simulink model "tcp_gantry_logic"  (R2025b)
settings: Solver=FixedStepAuto  StartTime=0.0  StopTime=inf  RelTol=1e-3  EnableMultiTasking=on
libraries: simulink x4, raspberrypiNetworklib x1
settings Model: ExtModeTrigDuration=2  Creator=rico_jitin  LastModifiedBy=rico_jitin
settings SolverCC: PositivePriorityOrder=on
settings OptimizationCC: EnhancedBackFolding=on  PassReuseOutputArgsAs=Individual arguments  ZeroExternalMemoryAtStartup=off  ZeroInternalMemoryAtStartup=off  MaxStackSize=200000  OptimizeBlockOrder=speed  DifferentSizesBufferReuse=on  OptimizationCustomize=off  EfficientTunableParamExpr=on
settings DebuggingCC: ParameterTunabilityLossMsg=error
settings HardwareCC: ProdBitPerPointer=32.0  ProdBitPerSizeT=32.0  ProdBitPerPtrDiffT=32.0  ProdLargestAtomicInteger=Long  ProdLargestAtomicFloat=Double  ProdWordSize=32.0  ProdLongLongMode=on  ProdHWDeviceType=ARM Compatible->ARM Cortex-A (32-bit)
settings RTWCC: SystemTargetFile=ert.tlc  HardwareBoard=Raspberry Pi  TLCOptions="-aInlineSetEventsForThisBaseRateFcn=TLC_FALSE -aSuppressMultiTaskScheduler=TLC_FALSE  -aRateBasedStepFcn=0"  TemplateMakefile=ert_default_tmf  Toolchain=GNU GCC Embedded Linux  BuildConfiguration=Faster Runs  Description=Embedded Coder
settings CodeAppCC: ForceParamTrailComments=on  IgnoreCustomStorageClasses=off  OperatorAnnotations=on  SimulinkDataObjDesc=on  SFDataObjDesc=on  InsertBlockDesc=on
settings ERTTargetCC: ExtModeTransport=2.0  ExtModeStaticAlloc=on  ExtModeMexFile=ext_xcp  ExtModeIntrfLevel=Level2 - Open  InlinedParameterPlacement=Hierarchical  CodeReplacementLibrary=ARM Cortex-A CMSIS  SupportVariableSizeSignals=on

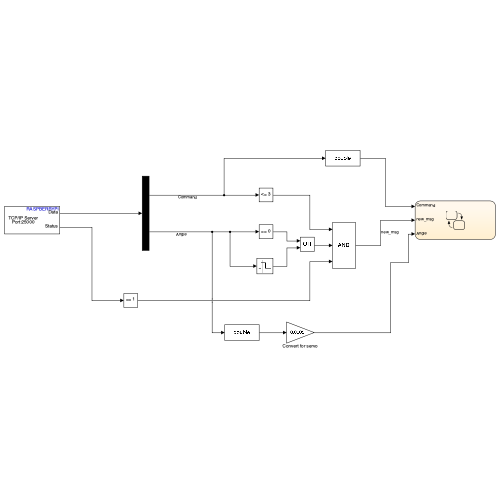
[thumbnail: Simulink's stored preview of the top-level diagram]
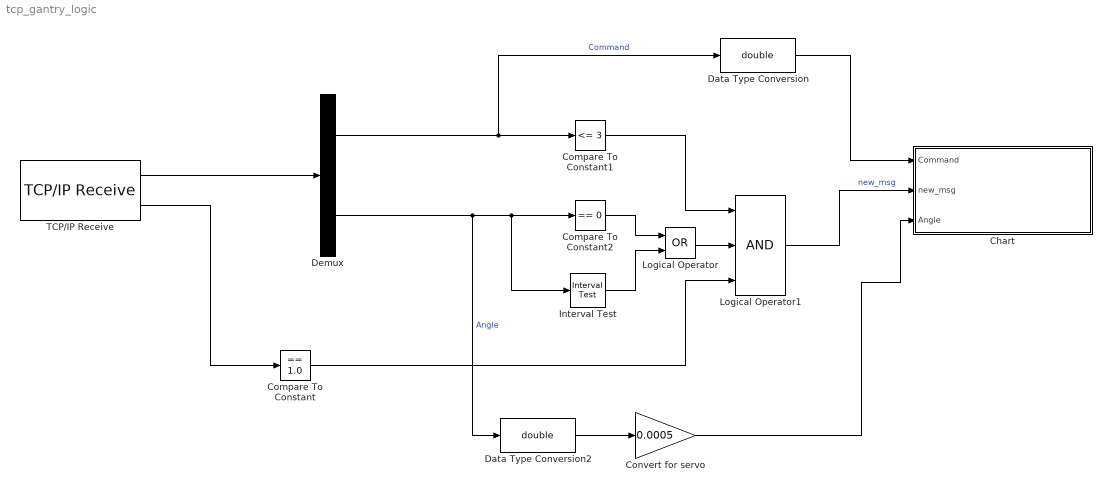
== system tcp_gantry_logic ==
  Chart : Stateflow chart  TreatAsAtomicUnit=on
  Compare To Constant : simulink/Logic and Bit Operations/Compare To Constant  relop===  const=1.0  OutDataTypeStr=boolean
  Compare To Constant1 : simulink/Logic and Bit Operations/Compare To Constant  relop=<=  const=3  OutDataTypeStr=boolean
  Compare To Constant2 : simulink/Logic and Bit Operations/Compare To Constant  relop===  const=0  OutDataTypeStr=boolean
  Convert for servo : Gain  Gain=0.0005
  Data Type Conversion : DataTypeConversion  OutDataTypeStr=double  SaturateOnIntegerOverflow=off  RndMeth=Floor
  Data Type Conversion2 : DataTypeConversion  OutDataTypeStr=double  SaturateOnIntegerOverflow=off  RndMeth=Floor
  Demux : Demux  Outputs=2
  Interval Test : simulink/Logic and Bit Operations/Interval Test  IntervalClosedRight=on  uplimit=200  IntervalClosedLeft=on  lowlimit=100  OutDataTypeStr=boolean
  Logical Operator : Logic  Operator=OR  AllPortsSameDT=off  OutDataTypeStr=boolean
  Logical Operator1 : Logic  Inputs=3  AllPortsSameDT=off  OutDataTypeStr=boolean
  TCP/IP Receive : raspberrypiNetworklib/TCP//IP Receive  Mode_=Server  LocalServerPort_=25000  RemoteAddr_=127.0.0.1  RemoteServerPort_=25000  DataType_=uint8  DataSize_=2  SampleTime_=0.002  SimulateUsing=Code generation  ClientPortBindingSelection_=off  ClientPortToBind_=35000  BlockingMode_=off  BlockTimeout_=0.1  BlockPlatform=RASPBERRYPI
  wires:
  TCP/IP Receive/1 -> Demux/1
  Demux/1 -> Data Type Conversion/1, Compare To Constant1/1  "Command"
  Demux/2 -> Data Type Conversion2/1, Interval Test/1, Compare To Constant2/1  "Angle"
  TCP/IP Receive/2 -> Compare To Constant/1
  Compare To Constant2/1 -> Logical Operator/1
  Interval Test/1 -> Logical Operator/2
  Logical Operator/1 -> Logical Operator1/2
  Compare To Constant1/1 -> Logical Operator1/1
  Compare To Constant/1 -> Logical Operator1/3
  Logical Operator1/1 -> Chart/2(new_msg)  "new_msg"
  Data Type Conversion2/1 -> Convert for servo/1
  Data Type Conversion/1 -> Chart/1(Command)
  Convert for servo/1 -> Chart/3(Angle)

== stateflow chart tcp_gantry_logic/Chart ==
  data: Command input; new_msg input; Angle input
